simulink library "casper_library_scopes"  (Simulink 8.0)
settings: Solver=ode45  SolverMode=SingleTasking  StartTime=0.0  StopTime=10.0  RelTol=1e-3
libraries: xbsIndex_r4 x476, xps_library x33, casper_library_misc x13, casper_library_scopes x5, casper_library_flow_control x1, simulink x1
(part 1 of 5)
settings Model: Creator=mdexter  LastModifiedBy=paulp

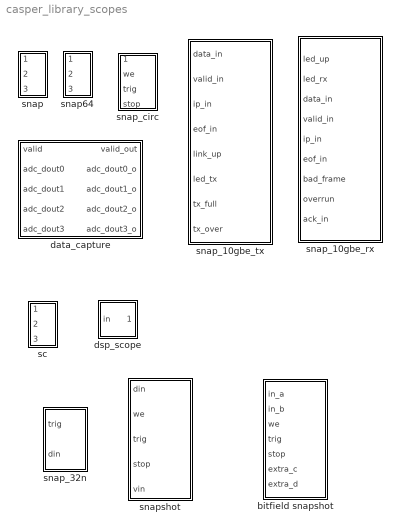
== system casper_library_scopes ==
  bitfield snapshot : Subsystem  Tag=casper:bitsnap  mask(bitsnap){io_names=[a b], io_widths=[16 1], io_bps=[14 0], io_types=[0 2], show_format=on, snap_storage=bram, snap_dram_dimm=2, snap_dram_clock=250, snap_nsamples=10, snap_data_width=32, snap_offset=on, snap_circap=on, snap_value=on, snap_use_dsp48=on, snap_delay=0, extra_names=[c d], extra_widths=[30 2], extra_bps=[0 0], extra_types=[0 0]}
      mask prompts: io_names "Names [msb...lsb]"; io_widths "Bitwidths [msb...lsb]"; io_bps "Binary pts [msb...lsb]"; io_types "Data types [msb...lsb], ufix=0, fix=1, bool=2"; show_format "Print format string?"; snap_storage "Storage medium"; snap_dram_dimm "DRAM dimm"; snap_dram_clock "DRAM clock rate"; snap_nsamples "Number of Samples (2^?)"; snap_data_width "Data width"; snap_offset "Start delay support"; snap_circap "Circular capture support"; snap_value "Extra value capture support"; snap_use_dsp48 "Use DSP48s to implement counters"; snap_delay "Pre-snapshot delay"; extra_names "Names [msb...lsb]"; extra_widths "Widths [msb...lsb]"; extra_bps "Binary pts [msb...lsb]"; extra_types "Data types [msb...lsb], ufix=0, fix=1, bool=2"
      mask help:
      | A wrapped snapshot block. Allows specification of inputs to a snapblock word so the toolflow can automatically set up the scope.
      | See documentation for snapshot for explanation of parameters.
      mask init:
      | bitsnap_init(gcb);
      settings: AttributesFormatString=snap(2):uf16.14,b\nextra(2):uf30.0,uf2.0
      mask TypeOptions snap_storage: bram | dram
      mask Callback snap_storage: bitsnap_callback();
      mask TypeOptions snap_dram_dimm: 1 | 2 | 3 | 4
      mask TypeOptions snap_dram_clock: 200 | 250 | 266 | 300 | 333
      mask TypeOptions snap_data_width: 8 | 16 | 32 | 64 | 128
      mask Callback snap_value: bitsnap_callback();
  data_capture : Subsystem  mask(data_capture){stream_name=adc_dout, nsimult_streams=4}
      mask prompts: stream_name "Stream Name"; nsimult_streams "Number Of Simultaneous Streams"
      mask help:
      | This block is useful for capturing parallel data streams
      | simultaneously and sending the data in structures for analysis
      | using MATLAB.  It is intended as a partial replacement for the
      | Simulink scope block when used with the functions in data_capture_tools.
      |
      | The block does not alter the data at all and costs no hardware
      | because it is purely a simulation block.  The block's Simulink
      | outputs are exactly the same as its inputs with no delay.
      mask init:
      | data_capture_init(gcb, ...
      |     'stream_name', stream_name, ...
      |     'nsimult_streams', nsimult_streams);
  dsp_scope : Subsystem  mask(dsp_scope){n_inputs=4, slice_width=18, bin_pt=17, arith_type=1}
      mask prompts: n_inputs "Number of inputs"; slice_width "Width of each input"; bin_pt "Output Binary Point"; arith_type "Output Arithmetic Type (0=Unsigned, 1 = Signed)"
      mask help:
      | This block provides a convenient interface to plotting waveforms
      | of blocks with serial data output in parallel.  The core example
      | is of the ADC, which outputs 8 samples / clock.  This scope (simulation only)
      | samples sufficently fast (based on the number of parallel inputs)
      | to serialize the output for view in a standard simulink scope.
      |
      | The input must be concatenated parallel data streams, and
      | each data binary point must be 0.  The easiest way to do this is
      | to push  all the inputs through a "cram" block from the
      | GAVRT blockset.
      | easy
      mask init:
      | dsp_scope_init(gcb, ...
      |     'n_inputs', n_inputs, ...
      |     'slice_width', slice_width, ...
      |     'bin_pt', bin_pt, ...
      |     'arith_type', arith_type);
  sc : Subsystem  mask(sc){nsamples=11, offset=0}
      mask prompts: nsamples "No. of samples(2^?)"; offset "Parallel Bus Offset"
      mask help:
      | The 'sc' block is a modified version of the 'snap' block in
      | the same library.  The modification intends to move the software
      | register which has partial control over the 'we' line to the
      | bram as an external port so that multiple brams can use the same
      | gated write enable, i.e. they can share the software register
      | that enables writing to the bram.  This will simplify synchronous writing
      | to multiple brams.
      |
      | The 'sc' core is used in the 'snap_32n' block to mask the
      | 32-bit word limitation of the bram.
      mask init:
      | deprecation_warning('the sc block is to be removed from the casper library, please use the snapshot block instead', 'sc');
      settings: CopyFcn=deprecation_warning('the sc block is to be removed from the casper library, please use the snapshot block instead', 'sc')
      mask Help: eval('xlWeb(''http://casper.berkeley.edu/wiki/Snap'')')
  snap : Subsystem  mask(snap){nsamples=11}
      mask prompts: nsamples "No. of samples(2^?)"
      mask help:
      | The <i>snap</i> block provides a packaged solution to capturing data from
      | the FPGA fabric and making it accessible from the CPU.  The block comes in
      | 2 flavors: <i>snap</i> (which captures to a 32 bit wide Shared BRAM), and
      | <i>snap64</i> (which captures to 2x32 bit wide Shared BRAMs to effect a
      | 64 bit capture).
      mask init:
      | deprecation_warning('the snap block is to be removed from the casper library, please use the snapshot block instead', 'snap');
      settings: CopyFcn=deprecation_warning('the snap block is to be removed from the casper library, please use the snapshot block instead', 'snap')
      mask Help: eval('xlWeb(''http://casper.berkeley.edu/wiki/Snap'')')
  snap64 : Subsystem  mask(snap64){nsamples=11}
      mask prompts: nsamples "No. of samples(2^?)"
      mask help:
      | The <i>snap</i> block provides a packaged solution to capturing data from
      | the FPGA fabric and making it accessible from the CPU.  The block comes in
      | 2 flavors: <i>snap</i> (which captures to a 32 bit wide Shared BRAM), and
      | <i>snap64</i> (which captures to 2x32 bit wide Shared BRAMs to effect a
      | 64 bit capture).
      mask init:
      | deprecation_warning('the snap64 block is to be removed from the casper library, please use the snapshot block instead', 'snap64');
      settings: CopyFcn=deprecation_warning('the snap64 block is to be removed from the casper library, please use the snapshot block instead', 'snap64')
      mask Help: eval('xlWeb(''http://casper.berkeley.edu/wiki/Snap'')')
  snap_10gbe_rx : Subsystem  mask(snap_10gbe_rx){nsamples=11}
      mask prompts: nsamples "No. of samples(2^?)"
      mask help:
      | This snap block provides a packaged solution to capturing a 10GbE datastream from the FPGA fabric and making it accessible from the CPU.  The block captures data in 3 32-bit brams, two for the main data stream and one for out-of-band data (IP addresses, link status, buffer overflow warnings etc).
      |
      | There are two versions, one tailored for RX data streams and one tailored for TX data streams.
      mask init:
      | deprecation_warning('the snap_10gbe_rx block is to be removed from the casper library, please use the snapshot block instead', 'snap_10gbe_rx');
      settings: CopyFcn=deprecation_warning('the snap_10gbe_rx block is to be removed from the casper library, please use the snapshot block instead', 'snap_10gbe_rx')
  snap_10gbe_tx : Subsystem  mask(snap_10gbe_tx){nsamples=11}
      mask prompts: nsamples "No. of samples(2^?)"
      mask help:
      | This snap block provides a packaged solution to capturing a 10GbE datastream from the FPGA fabric and making it accessible from the CPU.  The block captures data in 3 32-bit brams, two for the main data stream and one for out-of-band data (IP addresses, link status, buffer overflow warnings etc).
      |
      | There are two versions, one tailored for RX data streams and one tailored for TX data streams.
      mask init:
      | deprecation_warning('the snap_10gbe_tx block is to be removed from the casper library, please use the snapshot block instead', 'snap_10gbe_tx');
      settings: CopyFcn=deprecation_warning('the snap_10gbe_tx block is to be removed from the casper library, please use the snapshot block instead', 'snap_10gbe_tx')
  snap_32n : Subsystem  mask(snap_32n){nsamples=11, width=4}
      mask prompts: nsamples "Number of Samples (2^"; width "Input Bus Width (32x"
      mask help:
      | Like the snap64 block, this block contains multiple sub-cores
      | that each have a separate bram.  The purpose is to be able to
      | extend the functionality of the 'snap' and 'sc' blocks to beyond
      | the 32-bit word limitation of a single bram by synchronously
      | writing different parts of a larger bus to separate BRAMs.  UNLIKE
      | the snap64 block, the bus width on the 'snap_32n' block is
      | parameterizable to any multiple of 32.
      mask init:
      | deprecation_warning('The snap_32n block is to be removed from the casper library, please use the snapshot block instead', 'snap_32n');
      | snap_32n_init(gcb, ...
      |     'nsamples', nsamples, ...
      |     'width', width);
      settings: CopyFcn=deprecation_warning('the snap_32n block is to be removed from the casper library, please use the snapshot block instead', 'snap_32n')
  snap_circ : Subsystem  mask(snap_circ){nsamples=10}
      mask prompts: nsamples "Number of Samples (2^?)"
      mask help:
      | Backwards compatible with the normal snap block, but with the following upgrades:
      |  1) Ability to offset the trigger. Optionally delay the fabric trigger by a user-specified number of valids.
      |  2) 'Addr' register's MSb now indicates 'busy capturing'.
      |  3) Ability to capture continuously until a stop pulse is received. Data is captured into BRAM continuously, with old data being overwritten until a stop command is received. Then stop capturing when memory is filled. This enables you to get some data before and some data after the stop pulse. Use the 'tr_en_cnt' register to determine where you are in your vector.
      mask init:
      | deprecation_warning('the snap_circ block is to be removed from the casper library, please use the snapshot block instead', 'snap_circ');
      settings: CopyFcn=deprecation_warning('the snap_circ block is to be removed from the casper library, please use the snapshot block instead', 'snap_circ')
  snapshot : Subsystem  Tag=casper:snapshot  mask(snapshot){storage=bram, dram_dimm=1, dram_clock=200, nsamples=10, data_width=32, offset=on, circap=on, value=on, use_dsp48=on}
      mask prompts: storage "Storage medium"; dram_dimm "DRAM dimm"; dram_clock "DRAM clock rate"; nsamples "Number of Samples (2^?)"; data_width "Data width"; offset "Start delay support"; circap "Circular capture support"; value "Extra value capture support"; use_dsp48 "Use DSP48s to implement counters"
      mask help:
      | Standard snap block, but with the following optional extras;
      |  1) Optionally delay the fabric trigger by a user-specified number of valids.
      |  2) Capture continuously after a trigger until a stop pulse is received. Data is captured into BRAM continuously, with old data being overwritten until a stop command is received. Then stop capturing when memory is filled. This enables you to get some data before and some data after the stop pulse. Use the 'tr_en_cnt' register to determine where you are in your vector. 'Addr' register's MSb now indicates 'busy capturing'.
      |  3) Optionally capture a value on an input port to a register at the same time as the first data sample.
      |  4) Implement counters using DSP48Es to save resources.
      mask init:
      | snapshot_init(gcb, ...
      |     'storage', storage, ...
      |     'dram_dimm', dram_dimm, ...
      |     'dram_clock', dram_clock, ...
      |     'nsamples', nsamples, ...
      |     'data_width', data_width, ...
      |     'offset', offset, ...
      |     'circap', circap, ...
      |     'value', value, ...
      |     'use_dsp48', use_dsp48);
      mask TypeOptions storage: bram | dram
      mask Callback storage: snapshot_callback();
      mask TypeOptions dram_dimm: 1 | 2 | 3 | 4
      mask TypeOptions dram_clock: 200 | 250 | 266 | 300 | 333
      mask TypeOptions data_width: 8 | 16 | 32 | 64 | 128

== system casper_library_scopes/bitfield snapshot ==
  in_a : Inport
  in_b : Inport  Port=2
  we : Inport  Port=3
  trig : Inport  Port=4
  stop : Inport  Port=5
  extra_c : Inport  Port=6
  extra_d : Inport  Port=7
  assert_a : xbsIndex_r4/Assert  assert_type=on  type_source=Explicitly  gui_display_data_type=Fixed-point  arith_type=Unsigned  n_bits=16  bin_pt=14  preci_type=Single  exp_width=8  frac_width=24  assert_rate=off  rate_source=Explicitly  period=1  output_port=on  block_type=assert
  assert_b : xbsIndex_r4/Assert  assert_type=on  type_source=Explicitly  gui_display_data_type=Boolean  arith_type=Boolean  n_bits=1  bin_pt=0  preci_type=Single  exp_width=8  frac_width=24  assert_rate=off  rate_source=Explicitly  period=1  output_port=on  block_type=assert
  assextra_c : xbsIndex_r4/Assert  assert_type=on  type_source=Explicitly  gui_display_data_type=Fixed-point  arith_type=Unsigned  n_bits=30  bin_pt=0  preci_type=Single  exp_width=8  frac_width=24  assert_rate=off  rate_source=Explicitly  period=1  output_port=on  block_type=assert
  assextra_d : xbsIndex_r4/Assert  assert_type=on  type_source=Explicitly  gui_display_data_type=Fixed-point  arith_type=Unsigned  n_bits=2  bin_pt=0  preci_type=Single  exp_width=8  frac_width=24  assert_rate=off  rate_source=Explicitly  period=1  output_port=on  block_type=assert
  buscreate : Subsystem  AncestorBlock=casper_library_flow_control/bus_create  mask(bus_create){inputNum=2}
      mask prompts: inputNum "Number of inputs:"
      mask init:
      | bus_create_init(gcb,...
      |     'inputNum', inputNum);
  extracast : xbsIndex_r4/Convert  gui_display_data_type=Fixed-point  arith_type=Unsigned  n_bits=32  bin_pt=0  float_type=Single  exp_bits=8  fraction_bits=24  quantization=Truncate  overflow=Wrap  en=off  latency=0  dbl_ovrd=off  pipeline=off  block_type=convert
  extracreate : Subsystem  AncestorBlock=casper_library_flow_control/bus_create  mask(bus_create){inputNum=2}
      mask prompts: inputNum "Number of inputs:"
      mask init:
      | bus_create_init(gcb,...
      |     'inputNum', inputNum);
  ss : Subsystem  Tag=casper:snapshot  AncestorBlock=casper_library_scopes/snapshot  mask(snapshot){storage=bram, dram_dimm=2, dram_clock=250, nsamples=10, data_width=32, offset=on, circap=on, value=on, use_dsp48=on}
      mask prompts: storage "Storage medium"; dram_dimm "DRAM dimm"; dram_clock "DRAM clock rate"; nsamples "Number of Samples (2^?)"; data_width "Data width"; offset "Start delay support"; circap "Circular capture support"; value "Extra value capture support"; use_dsp48 "Use DSP48s to implement counters"
      mask help:
      | Standard snap block, but with the following optional extras;
      |  1) Optionally delay the fabric trigger by a user-specified number of valids.
      |  2) Capture continuously after a trigger until a stop pulse is received. Data is captured into BRAM continuously, with old data being overwritten until a stop command is received. Then stop capturing when memory is filled. This enables you to get some data before and some data after the stop pulse. Use the 'tr_en_cnt' register to determine where you are in your vector. 'Addr' register's MSb now indicates 'busy capturing'.
      |  3) Optionally capture a value on an input port to a register at the same time as the first data sample.
      |  4) Implement counters using DSP48Es to save resources.
      mask init: same as casper_library_scopes/snapshot
      mask TypeOptions storage: bram | dram
      mask Callback storage: snapshot_callback();
      mask TypeOptions dram_dimm: 1 | 2 | 3 | 4
      mask TypeOptions dram_clock: 200 | 250 | 266 | 300 | 333
      mask TypeOptions data_width: 8 | 16 | 32 | 64 | 128
  wires:
  buscreate/1(bus_out) -> ss/1(din)
  in_a/1 -> assert_a/1
  assert_a/1 -> buscreate/1(in1)
  in_b/1 -> assert_b/1
  assert_b/1 -> buscreate/2(in2)
  we/1 -> ss/2(we)
  trig/1 -> ss/3(trig)
  stop/1 -> ss/4(stop)
  extracreate/1(bus_out) -> extracast/1
  extracast/1 -> ss/5(vin)
  extra_c/1 -> assextra_c/1
  assextra_c/1 -> extracreate/1(in1)
  extra_d/1 -> assextra_d/1
  assextra_d/1 -> extracreate/2(in2)

== system casper_library_scopes/data_capture ==
  valid : Inport
  adc_dout0 : Inport  Port=2
  adc_dout1 : Inport  Port=3
  adc_dout2 : Inport  Port=4
  adc_dout3 : Inport  Port=5
  ToWorkspace_adc_dout0 : ToWorkspace  VariableName=adc_dout0  SampleTime=-1  SaveFormat=Structure
  ToWorkspace_adc_dout1 : ToWorkspace  VariableName=adc_dout1  SampleTime=-1  SaveFormat=Structure
  ToWorkspace_adc_dout2 : ToWorkspace  VariableName=adc_dout2  SampleTime=-1  SaveFormat=Structure
  ToWorkspace_adc_dout3 : ToWorkspace  VariableName=adc_dout3  SampleTime=-1  SaveFormat=Structure
  ToWorkspace_valid : ToWorkspace  VariableName=adc_dout_valid  SampleTime=-1  SaveFormat=Structure
  valid_out : Outport
  adc_dout0_o : Outport  Port=2
  adc_dout1_o : Outport  Port=3
  adc_dout2_o : Outport  Port=4
  adc_dout3_o : Outport  Port=5
  wires:
  adc_dout3/1 -> adc_dout3_o/1, ToWorkspace_adc_dout3/1
  adc_dout2/1 -> adc_dout2_o/1, ToWorkspace_adc_dout2/1
  adc_dout1/1 -> adc_dout1_o/1, ToWorkspace_adc_dout1/1
  adc_dout0/1 -> adc_dout0_o/1, ToWorkspace_adc_dout0/1
  valid/1 -> valid_out/1, ToWorkspace_valid/1

== system casper_library_scopes/dsp_scope ==
  in : Inport
  bus_expand : casper_library_flow_control/bus_expand  mode=divisions of equal size  outputNum=4  outputWidth=18  outputBinaryPt=17  outputArithmeticType=1  show_format=off  outputToWorkspace=off  variablePrefix=out  outputToModelAsWell=on
      settings: AttributesFormatString=4 outputs
  sel : simulink/Sources/Counter Free-Running  NumBits=2  tsamp=0.25
  switch : MultiPortSwitch  DataPortOrder=Zero-based contiguous  Inputs=4  zeroidx=on
  out : Outport
  wires:
  in/1 -> bus_expand/1
  switch/1 -> out/1
  sel/1 -> switch/1
  bus_expand/1 -> switch/2
  bus_expand/2 -> switch/3
  ? -> switch/4
  ? -> switch/5

== system casper_library_scopes/sc ==
  din : Inport
  trig : Inport  Port=2
  read_freeze : Inport  Port=3
  Constant : xbsIndex_r4/Constant  const=2^nsamples  gui_display_data_type=Fixed-point  arith_type=Unsigned  n_bits=32  bin_pt=0  preci_type=Single  exp_width=8  frac_width=24  explicit_period=on  period=1  equ=P=C  opselect=C  inp2=PCIN>>17  opr=+  inp1=P  carry=CIN  dbl_ovrd=off  block_type=constant
  Counter : xbsIndex_r4/Counter  cnt_type=Count Limited  cnt_to=Inf  operation=Up  start_count=0  cnt_by_val=1  arith_type=Unsigned  n_bits=nsamples+1  bin_pt=0  load_pin=off  rst=on  en=off  explicit_period=on  period=1  dbl_ovrd=off  use_behavioral_HDL=off  implementation=Fabric  use_rpm=off  block_type=counter
  Inverter : xbsIndex_r4/Inverter  en=off  latency=0  dbl_ovrd=off  block_type=inv
  Logical : xbsIndex_r4/Logical  logical_function=AND  inputs=2  en=off  latency=0  precision=Full  arith_type=Unsigned  n_bits=16  bin_pt=0  align_bp=on  dbl_ovrd=off  block_type=logical
  Reinterpret : xbsIndex_r4/Reinterpret  force_arith_type=on  arith_type=Unsigned  force_bin_pt=on  bin_pt=0  block_type=reinterpret
      settings: infoedit="Changes signal type without altering the binary representation.   You can changed the signal between signed and unsigned, and relocate the binary point.<P><P>Hardware notes: In hardware this block costs nothing.<P><P>Example:  Suppose the input is 6 bits wide, signed, with 2 fractional bits, and the output is forced to unsigned with 0 fractional bits.  Then an input of -2.0 (1110.00 in binary 2's complement) becomes an output of 56 (111000 in binary)."  block_version=10.1.1
  Relational : xbsIndex_r4/Relational  mode=a<b  en=off  latency=1  dbl_ovrd=off  block_type=relational
      settings: block_version=10.1.3
  Slice : xbsIndex_r4/Slice  nbits=1  boolean_output=on  mode=Lower Bit Location + Width  bit1=0  base1=MSB of Input  bit0=0  base0=LSB of Input  dbl_ovrd=off  block_type=slice
      settings: infoedit="Extracts a given range of bits from each input sample and presents it at the output.  The output type is ordinarily unsigned with binary point at zero, but can be Boolean when the slice is one bit wide.<P><P>Hardware notes: In hardware this block costs nothing."  block_version=10.1.3
  bram : xps_library/Shared BRAM  Tag=xps:bram  arith_type=Unsigned  addr_width=nsamples  data_width=32  reg_prim_output=on  reg_core_output=on  optimization=Minimum_Area  data_bin_pt=0  init_vals=0  sample_rate=1
  data_sl : xbsIndex_r4/Slice  nbits=32  boolean_output=off  mode=Lower Bit Location + Width  bit1=0  base1=MSB of Input  bit0=offset  base0=LSB of Input  dbl_ovrd=off  block_type=slice
      settings: infoedit="Extracts a given range of bits from each input sample and presents it at the output.  The output type is ordinarily unsigned with binary point at zero, but can be Boolean when the slice is one bit wide.<P><P>Hardware notes: In hardware this block costs nothing."  block_version=10.1.3
  wires:
  data_sl/1 -> Reinterpret/1
  Constant/1 -> Relational/2
  Relational/1 -> bram/3
  read_freeze/1 -> Slice/1
  Slice/1 -> Inverter/1
  Logical/1 -> Counter/1
  Inverter/1 -> Logical/2
  trig/1 -> Logical/1
  Counter/1 -> Relational/1, bram/1
  Reinterpret/1 -> bram/2
  din/1 -> data_sl/1

== system casper_library_scopes/snap ==
  din : Inport
  trig : Inport  Port=2
  we : Inport  Port=3
  Constant : xbsIndex_r4/Constant  const=1  gui_display_data_type=Fixed-point  arith_type=Boolean  n_bits=1  bin_pt=0  preci_type=Single  exp_width=8  frac_width=24  explicit_period=on  period=1  equ=P=C  opselect=C  inp2=PCIN>>17  opr=+  inp1=P  carry=CIN  dbl_ovrd=off  block_type=constant
      settings: block_version=10.1.1
  Constant1 : xbsIndex_r4/Constant  const=1  gui_display_data_type=Fixed-point  arith_type=Boolean  n_bits=1  bin_pt=0  preci_type=Single  exp_width=8  frac_width=24  explicit_period=on  period=1  equ=P=C  opselect=C  inp2=PCIN>>17  opr=+  inp1=P  carry=CIN  dbl_ovrd=off  block_type=constant
      settings: block_version=10.1.1
  Constant13 : Constant
  Constant2 : xbsIndex_r4/Constant  const=1  gui_display_data_type=Fixed-point  arith_type=Boolean  n_bits=1  bin_pt=0  preci_type=Single  exp_width=8  frac_width=24  explicit_period=on  period=1  equ=P=C  opselect=C  inp2=PCIN>>17  opr=+  inp1=P  carry=CIN  dbl_ovrd=off  block_type=constant
      settings: block_version=10.1.1
  Inverter : xbsIndex_r4/Inverter  en=off  latency=0  dbl_ovrd=off  block_type=inv
      settings: xl_area=[0, 0, 0, 0, 0, 0, 0]  block_version=10.1.1
  Logical1 : xbsIndex_r4/Logical  logical_function=AND  inputs=2  en=off  latency=0  precision=Full  arith_type=Unsigned  n_bits=8  bin_pt=2  align_bp=on  dbl_ovrd=off  block_type=logical
      settings: xl_area=[0, 0, 0, 0, 0, 0, 0]  block_version=10.1.1
  Mux1 : xbsIndex_r4/Mux  inputs=2  en=off  latency=0  precision=Full  arith_type="Signed  (2's comp)"  n_bits=8  bin_pt=2  quantization=Truncate  overflow=Wrap  dbl_ovrd=off  block_type=mux
      settings: xl_area=[0, 0, 0, 0, 0, 0, 0]  block_version=10.1.1
  Mux2 : xbsIndex_r4/Mux  inputs=2  en=off  latency=0  precision=Full  arith_type="Signed  (2's comp)"  n_bits=8  bin_pt=2  quantization=Truncate  overflow=Wrap  dbl_ovrd=off  block_type=mux
      settings: xl_area=[0, 0, 0, 0, 0, 0, 0]  block_version=10.1.1
  Register : xbsIndex_r4/Register  init=0  rst=on  en=on  dbl_ovrd=off  block_type=register
      settings: xl_area=[0, 0, 0, 0, 0, 0, 0]  block_version=10.1.1
  Register1 : xbsIndex_r4/Register  init=0  rst=on  en=on  dbl_ovrd=off  block_type=register
      settings: xl_area=[0, 0, 0, 0, 0, 0, 0]  block_version=10.1.1
  Reinterpret : xbsIndex_r4/Reinterpret  force_arith_type=on  arith_type=Unsigned  force_bin_pt=on  bin_pt=0  block_type=reinterpret
      settings: infoedit="Changes signal type without altering the binary representation.   You can changed the signal between signed and unsigned, and relocate the binary point.<P><P>Hardware notes: In hardware this block costs nothing.<P><P>Example:  Suppose the input is 6 bits wide, signed, with 2 fractional bits, and the output is forced to unsigned with 0 fractional bits.  Then an input of -2.0 (1110.00 in binary 2's complement) becomes an output of 56 (111000 in binary)."  block_version=10.1.1
  addr : xps_library/software register  Tag=xps:sw_reg  numios=1  io_dir=To Processor  io_delay=0  sample_period=1  name1=reg  bitwidth1=32  arith_type1=Unsigned  bin_pt1=0
  bram : xps_library/Shared BRAM  Tag=xps:bram  arith_type=Unsigned  addr_width=nsamples  data_width=32  reg_prim_output=on  reg_core_output=on  optimization=Minimum_Area  data_bin_pt=0  init_vals=0  sample_rate=1
  ctrl : xps_library/software register  Tag=xps:sw_reg  numios=1  io_dir=From Processor  io_delay=0  sample_period=1  name1=reg  bitwidth1=32  arith_type1=Unsigned  bin_pt1=0
  enable : xbsIndex_r4/Slice  nbits=1  boolean_output=on  mode=Lower Bit Location + Width  bit1=0  base1=LSB of Input  bit0=0  base0=LSB of Input  dbl_ovrd=off  block_type=slice
      settings: infoedit="Extracts a given range of bits from each input sample and presents it at the output.  The output type is ordinarily unsigned with binary point at zero, but can be Boolean when the slice is one bit wide.<P><P>Hardware notes: In hardware this block costs nothing."  block_version=10.1.1
  freeze_cntr : casper_library_misc/freeze_cntr  CounterBits=nsamples
  posedge : casper_library_misc/edge_detect  edge=Rising  polarity=Active High  x_in=[0 0.08 0.08 0.16 0.16 0.24 0.24 0.32 0.32 0.4]  y_in="[-1 -1  1  1  1  1  1  1  1  1]"  x_out=[0.6 0.68 0.68 0.76 0.76 0.84 0.84 0.92 0.92 1]  y_out="[-1 -1  1  1 -1 -1 -1 -1 -1 -1]"
  trig1 : xbsIndex_r4/Slice  nbits=1  boolean_output=on  mode=Lower Bit Location + Width  bit1=0  base1=LSB of Input  bit0=1  base0=LSB of Input  dbl_ovrd=off  block_type=slice
      settings: infoedit="Extracts a given range of bits from each input sample and presents it at the output.  The output type is ordinarily unsigned with binary point at zero, but can be Boolean when the slice is one bit wide.<P><P>Hardware notes: In hardware this block costs nothing."  block_version=10.1.1
  valid : xbsIndex_r4/Slice  nbits=1  boolean_output=on  mode=Lower Bit Location + Width  bit1=0  base1=LSB of Input  bit0=2  base0=LSB of Input  dbl_ovrd=off  block_type=slice
      settings: infoedit="Extracts a given range of bits from each input sample and presents it at the output.  The output type is ordinarily unsigned with binary point at zero, but can be Boolean when the slice is one bit wide.<P><P>Hardware notes: In hardware this block costs nothing."  block_version=10.1.1
  wires:
  Mux2/1 -> Logical1/1
  Inverter/1 -> Logical1/2
  Logical1/1 -> Register/2
  valid/1 -> Mux1/1
  trig1/1 -> Mux2/1
  Register1/1 -> addr/1
  Constant2/1 -> Mux1/3
  we/1 -> Mux1/2
  Mux1/1 -> freeze_cntr/1
  Constant1/1 -> Mux2/3
  Constant/1 -> Register/1
  posedge/1 -> Inverter/1, Register1/2, Register/3
  ctrl/1 -> trig1/1, valid/1, enable/1
  din/1 -> Reinterpret/1
  Reinterpret/1 -> bram/2
  Constant13/1 -> ctrl/1
  freeze_cntr/2 -> Register1/3, bram/3
  Register/1 -> freeze_cntr/2
  enable/1 -> posedge/1
  freeze_cntr/1 -> bram/1, Register1/1
  trig/1 -> Mux2/2

== system casper_library_scopes/snap64 ==
  din : Inport
  trig : Inport  Port=2
  we : Inport  Port=3
  Constant : xbsIndex_r4/Constant  const=1  gui_display_data_type=Fixed-point  arith_type=Boolean  n_bits=1  bin_pt=0  preci_type=Single  exp_width=8  frac_width=24  explicit_period=on  period=1  equ=P=C  opselect=C  inp2=PCIN>>17  opr=+  inp1=P  carry=CIN  dbl_ovrd=off  block_type=constant
      settings: block_version=10.1.1
  Constant1 : xbsIndex_r4/Constant  const=1  gui_display_data_type=Fixed-point  arith_type=Boolean  n_bits=1  bin_pt=0  preci_type=Single  exp_width=8  frac_width=24  explicit_period=on  period=1  equ=P=C  opselect=C  inp2=PCIN>>17  opr=+  inp1=P  carry=CIN  dbl_ovrd=off  block_type=constant
      settings: block_version=10.1.1
  Constant13 : Constant
  Constant2 : xbsIndex_r4/Constant  const=1  gui_display_data_type=Fixed-point  arith_type=Boolean  n_bits=1  bin_pt=0  preci_type=Single  exp_width=8  frac_width=24  explicit_period=on  period=1  equ=P=C  opselect=C  inp2=PCIN>>17  opr=+  inp1=P  carry=CIN  dbl_ovrd=off  block_type=constant
      settings: block_version=10.1.1
  Inverter : xbsIndex_r4/Inverter  en=off  latency=0  dbl_ovrd=off  block_type=inv
      settings: xl_area=[0, 0, 0, 0, 0, 0, 0]  block_version=10.1.1
  Logical1 : xbsIndex_r4/Logical  logical_function=AND  inputs=2  en=off  latency=0  precision=Full  arith_type=Unsigned  n_bits=8  bin_pt=2  align_bp=on  dbl_ovrd=off  block_type=logical
      settings: xl_area=[0, 0, 0, 0, 0, 0, 0]  block_version=10.1.1
  Mux1 : xbsIndex_r4/Mux  inputs=2  en=off  latency=0  precision=Full  arith_type="Signed  (2's comp)"  n_bits=8  bin_pt=2  quantization=Truncate  overflow=Wrap  dbl_ovrd=off  block_type=mux
      settings: xl_area=[0, 0, 0, 0, 0, 0, 0]  block_version=10.1.1
  Mux2 : xbsIndex_r4/Mux  inputs=2  en=off  latency=0  precision=Full  arith_type="Signed  (2's comp)"  n_bits=8  bin_pt=2  quantization=Truncate  overflow=Wrap  dbl_ovrd=off  block_type=mux
      settings: xl_area=[0, 0, 0, 0, 0, 0, 0]  block_version=10.1.1
  Register : xbsIndex_r4/Register  init=0  rst=on  en=on  dbl_ovrd=off  block_type=register
      settings: xl_area=[0, 0, 0, 0, 0, 0, 0]  block_version=10.1.1
  Register1 : xbsIndex_r4/Register  init=0  rst=on  en=on  dbl_ovrd=off  block_type=register
      settings: xl_area=[0, 0, 0, 0, 0, 0, 0]  block_version=10.1.1
  Reinterpret3 : xbsIndex_r4/Reinterpret  force_arith_type=on  arith_type=Unsigned  force_bin_pt=on  bin_pt=0  block_type=reinterpret
      settings: infoedit="Changes signal type without altering the binary representation.   You can changed the signal between signed and unsigned, and relocate the binary point.<P><P>Hardware notes: In hardware this block costs nothing.<P><P>Example:  Suppose the input is 6 bits wide, signed, with 2 fractional bits, and the output is forced to unsigned with 0 fractional bits.  Then an input of -2.0 (1110.00 in binary 2's complement) becomes an output of 56 (111000 in binary)."  block_version=10.1.1
  addr : xps_library/software register  Tag=xps:sw_reg  numios=1  io_dir=To Processor  io_delay=0  sample_period=1  name1=reg  bitwidth1=32  arith_type1=Unsigned  bin_pt1=0
  bram_lsb : xps_library/Shared BRAM  Tag=xps:bram  arith_type=Unsigned  addr_width=nsamples  data_width=32  reg_prim_output=on  reg_core_output=on  optimization=Minimum_Area  data_bin_pt=0  init_vals=0  sample_rate=1
  bram_msb : xps_library/Shared BRAM  Tag=xps:bram  arith_type=Unsigned  addr_width=nsamples  data_width=32  reg_prim_output=on  reg_core_output=on  optimization=Minimum_Area  data_bin_pt=0  init_vals=0  sample_rate=1
  ctrl : xps_library/software register  Tag=xps:sw_reg  numios=1  io_dir=From Processor  io_delay=0  sample_period=1  name1=reg  bitwidth1=32  arith_type1=Unsigned  bin_pt1=0
  en1 : xbsIndex_r4/Slice  nbits=32  boolean_output=off  mode=Lower Bit Location + Width  bit1=0  base1=LSB of Input  bit0=32  base0=LSB of Input  dbl_ovrd=off  block_type=slice
      settings: infoedit="Extracts a given range of bits from each input sample and presents it at the output.  The output type is ordinarily unsigned with binary point at zero, but can be Boolean when the slice is one bit wide.<P><P>Hardware notes: In hardware this block costs nothing."  block_version=10.1.1
  en2 : xbsIndex_r4/Slice  nbits=32  boolean_output=off  mode=Lower Bit Location + Width  bit1=0  base1=LSB of Input  bit0=0  base0=LSB of Input  dbl_ovrd=off  block_type=slice
      settings: infoedit="Extracts a given range of bits from each input sample and presents it at the output.  The output type is ordinarily unsigned with binary point at zero, but can be Boolean when the slice is one bit wide.<P><P>Hardware notes: In hardware this block costs nothing."  block_version=10.1.1
  enable : xbsIndex_r4/Slice  nbits=1  boolean_output=on  mode=Lower Bit Location + Width  bit1=0  base1=LSB of Input  bit0=0  base0=LSB of Input  dbl_ovrd=off  block_type=slice
      settings: infoedit="Extracts a given range of bits from each input sample and presents it at the output.  The output type is ordinarily unsigned with binary point at zero, but can be Boolean when the slice is one bit wide.<P><P>Hardware notes: In hardware this block costs nothing."  block_version=10.1.1
  freeze_cntr : casper_library_misc/freeze_cntr  CounterBits=nsamples
  posedge : casper_library_misc/edge_detect  edge=Rising  polarity=Active High  x_in=[0 0.08 0.08 0.16 0.16 0.24 0.24 0.32 0.32 0.4]  y_in="[-1 -1  1  1  1  1  1  1  1  1]"  x_out=[0.6 0.68 0.68 0.76 0.76 0.84 0.84 0.92 0.92 1]  y_out="[-1 -1  1  1 -1 -1 -1 -1 -1 -1]"
  trig1 : xbsIndex_r4/Slice  nbits=1  boolean_output=on  mode=Lower Bit Location + Width  bit1=0  base1=LSB of Input  bit0=1  base0=LSB of Input  dbl_ovrd=off  block_type=slice
      settings: infoedit="Extracts a given range of bits from each input sample and presents it at the output.  The output type is ordinarily unsigned with binary point at zero, but can be Boolean when the slice is one bit wide.<P><P>Hardware notes: In hardware this block costs nothing."  block_version=10.1.1
  valid : xbsIndex_r4/Slice  nbits=1  boolean_output=on  mode=Lower Bit Location + Width  bit1=0  base1=LSB of Input  bit0=2  base0=LSB of Input  dbl_ovrd=off  block_type=slice
      settings: infoedit="Extracts a given range of bits from each input sample and presents it at the output.  The output type is ordinarily unsigned with binary point at zero, but can be Boolean when the slice is one bit wide.<P><P>Hardware notes: In hardware this block costs nothing."  block_version=10.1.1
  wires:
  freeze_cntr/1 -> bram_lsb/1, bram_msb/1, Register1/1
  Register/1 -> freeze_cntr/2
  Mux2/1 -> Logical1/1
  Inverter/1 -> Logical1/2
  Logical1/1 -> Register/2
  valid/1 -> Mux1/1
  trig1/1 -> Mux2/1
  Register1/1 -> addr/1
  Constant2/1 -> Mux1/3
  we/1 -> Mux1/2
  Mux1/1 -> freeze_cntr/1
  Constant1/1 -> Mux2/3
  Constant/1 -> Register/1
  posedge/1 -> Inverter/1, Register1/2, Register/3
  ctrl/1 -> trig1/1, valid/1, enable/1
  Constant13/1 -> ctrl/1
  freeze_cntr/2 -> bram_lsb/3, bram_msb/3, Register1/3
  enable/1 -> posedge/1
  trig/1 -> Mux2/2
  Reinterpret3/1 -> en1/1, en2/1
  din/1 -> Reinterpret3/1
  en1/1 -> bram_msb/2
  en2/1 -> bram_lsb/2

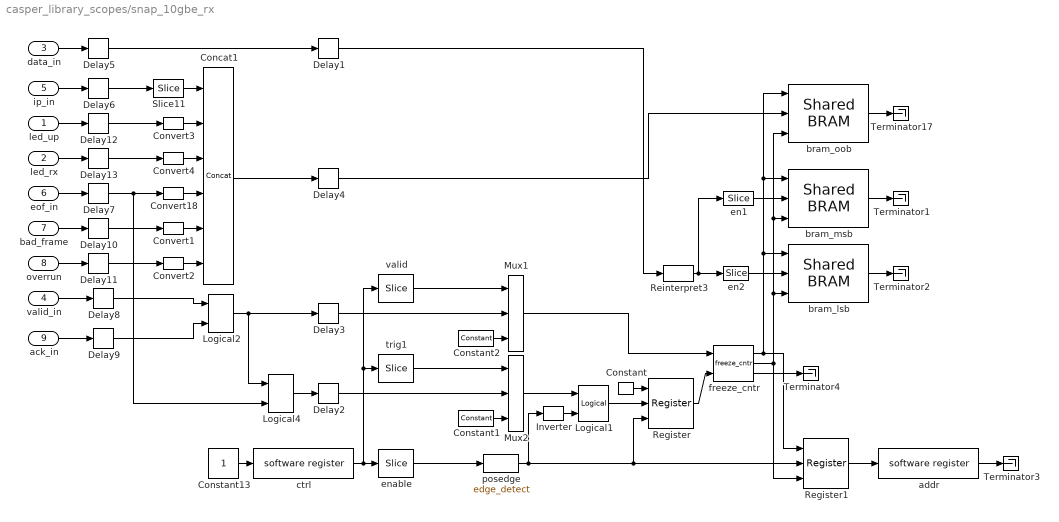
== system casper_library_scopes/snap_10gbe_rx ==
  led_up : Inport
  led_rx : Inport  Port=2
  data_in : Inport  Port=3
  valid_in : Inport  Port=4
  ip_in : Inport  Port=5
  eof_in : Inport  Port=6
  bad_frame : Inport  Port=7
  overrun : Inport  Port=8
  ack_in : Inport  Port=9
  Concat1 : xbsIndex_r4/Concat  num_inputs=6  dbl_ovrd=off  block_type=concat
      settings: block_version=10.1.3
  Constant : xbsIndex_r4/Constant  const=1  gui_display_data_type=Fixed-point  arith_type=Boolean  n_bits=1  bin_pt=0  preci_type=Single  exp_width=8  frac_width=24  explicit_period=on  period=1  equ=P=C  opselect=C  inp2=PCIN>>17  opr=+  inp1=P  carry=CIN  dbl_ovrd=off  block_type=constant
  Constant1 : xbsIndex_r4/Constant  const=1  gui_display_data_type=Fixed-point  arith_type=Boolean  n_bits=1  bin_pt=0  preci_type=Single  exp_width=8  frac_width=24  explicit_period=on  period=1  equ=P=C  opselect=C  inp2=PCIN>>17  opr=+  inp1=P  carry=CIN  dbl_ovrd=off  block_type=constant
  Constant13 : Constant
  Constant2 : xbsIndex_r4/Constant  const=1  gui_display_data_type=Fixed-point  arith_type=Boolean  n_bits=1  bin_pt=0  preci_type=Single  exp_width=8  frac_width=24  explicit_period=on  period=1  equ=P=C  opselect=C  inp2=PCIN>>17  opr=+  inp1=P  carry=CIN  dbl_ovrd=off  block_type=constant
  Convert{1..4,18} (5 alike) : xbsIndex_r4/Convert  gui_display_data_type=Fixed-point  arith_type=Unsigned  n_bits=1  bin_pt=0  float_type=Single  exp_bits=8  fraction_bits=24  quantization=Truncate  overflow=Wrap  en=off  latency=0  dbl_ovrd=off  pipeline=off  block_type=convert
      settings: xl_area=[0, 0, 0, 0, 0, 0, 0]  block_version=10.1.3
  Delay{1..13} (13 alike) : xbsIndex_r4/Delay  rst=off  infoeditControl=Selection of Reset will increase slice count due to use of real FFs and instead of SRLs  en=off  latency=2  dbl_ovrd=off  reg_retiming=on  block_type=delay
      settings: xl_area=[0, 0, 0, 0, 0, 0, 0]
  Inverter : xbsIndex_r4/Inverter  en=off  latency=0  dbl_ovrd=off  block_type=inv
      settings: xl_area=[0, 0, 0, 0, 0, 0, 0]
  Logical1 : xbsIndex_r4/Logical  logical_function=AND  inputs=2  en=off  latency=0  precision=Full  arith_type=Unsigned  n_bits=8  bin_pt=2  align_bp=on  dbl_ovrd=off  block_type=logical
      settings: xl_area=[0, 0, 0, 0, 0, 0, 0]
  Logical2 : xbsIndex_r4/Logical  logical_function=AND  inputs=2  en=off  latency=0  precision=Full  arith_type=Unsigned  n_bits=8  bin_pt=2  align_bp=on  dbl_ovrd=off  block_type=logical
      settings: xl_area=[0, 0, 0, 0, 0, 0, 0]
  Logical4 : xbsIndex_r4/Logical  logical_function=AND  inputs=2  en=off  latency=0  precision=Full  arith_type=Unsigned  n_bits=8  bin_pt=2  align_bp=on  dbl_ovrd=off  block_type=logical
      settings: xl_area=[0, 0, 0, 0, 0, 0, 0]
  Mux1 : xbsIndex_r4/Mux  inputs=2  en=off  latency=0  precision=Full  arith_type="Signed  (2's comp)"  n_bits=8  bin_pt=2  quantization=Truncate  overflow=Wrap  dbl_ovrd=off  block_type=mux
      settings: xl_area=[0, 0, 0, 0, 0, 0, 0]
  Mux2 : xbsIndex_r4/Mux  inputs=2  en=off  latency=0  precision=Full  arith_type="Signed  (2's comp)"  n_bits=8  bin_pt=2  quantization=Truncate  overflow=Wrap  dbl_ovrd=off  block_type=mux
      settings: xl_area=[0, 0, 0, 0, 0, 0, 0]
  Register : xbsIndex_r4/Register  init=0  rst=on  en=on  dbl_ovrd=off  block_type=register
      settings: xl_area=[0, 0, 0, 0, 0, 0, 0]
  Register1 : xbsIndex_r4/Register  init=0  rst=on  en=on  dbl_ovrd=off  block_type=register
      settings: xl_area=[0, 0, 0, 0, 0, 0, 0]
  Reinterpret3 : xbsIndex_r4/Reinterpret  force_arith_type=on  arith_type=Unsigned  force_bin_pt=on  bin_pt=0  block_type=reinterpret
      settings: infoedit="Changes signal type without altering the binary representation.   You can changed the signal between signed and unsigned, and relocate the binary point.<P><P>Hardware notes: In hardware this block costs nothing.<P><P>Example:  Suppose the input is 6 bits wide, signed, with 2 fractional bits, and the output is forced to unsigned with 0 fractional bits.  Then an input of -2.0 (1110.00 in binary 2's complement) becomes an output of 56 (111000 in binary)."  block_version=10.1.3
  Slice11 : xbsIndex_r4/Slice  nbits=32-5  boolean_output=off  mode=Lower Bit Location + Width  bit1=0  base1=MSB of Input  bit0=0  base0=LSB of Input  dbl_ovrd=off  block_type=slice
      settings: infoedit="Extracts a given range of bits from each input sample and presents it at the output.  The output type is ordinarily unsigned with binary point at zero, but can be Boolean when the slice is one bit wide.<P><P>Hardware notes: In hardware this block costs nothing."  block_version=10.1.3
  Terminator{1..4,17} (5 alike) : Terminator
  addr : xps_library/software register  Tag=xps:sw_reg  numios=1  io_dir=To Processor  io_delay=0  sample_period=1  name1=reg  bitwidth1=32  arith_type1=Unsigned  bin_pt1=0
  bram_lsb : xps_library/Shared BRAM  Tag=xps:bram  arith_type=Unsigned  addr_width=nsamples  data_width=32  reg_prim_output=on  reg_core_output=on  optimization=Minimum_Area  data_bin_pt=0  init_vals=0  sample_rate=1
  bram_msb : xps_library/Shared BRAM  Tag=xps:bram  arith_type=Unsigned  addr_width=nsamples  data_width=32  reg_prim_output=on  reg_core_output=on  optimization=Minimum_Area  data_bin_pt=0  init_vals=0  sample_rate=1
  bram_oob : xps_library/Shared BRAM  Tag=xps:bram  arith_type=Unsigned  addr_width=nsamples  data_width=32  reg_prim_output=on  reg_core_output=on  optimization=Minimum_Area  data_bin_pt=0  init_vals=0  sample_rate=1
  ctrl : xps_library/software register  Tag=xps:sw_reg  numios=1  io_dir=From Processor  io_delay=0  sample_period=1  name1=reg  bitwidth1=32  arith_type1=Unsigned  bin_pt1=0
  en1 : xbsIndex_r4/Slice  nbits=32  boolean_output=off  mode=Lower Bit Location + Width  bit1=0  base1=LSB of Input  bit0=32  base0=LSB of Input  dbl_ovrd=off  block_type=slice
      settings: infoedit="Extracts a given range of bits from each input sample and presents it at the output.  The output type is ordinarily unsigned with binary point at zero, but can be Boolean when the slice is one bit wide.<P><P>Hardware notes: In hardware this block costs nothing."  block_version=10.1.3
  en2 : xbsIndex_r4/Slice  nbits=32  boolean_output=off  mode=Lower Bit Location + Width  bit1=0  base1=LSB of Input  bit0=0  base0=LSB of Input  dbl_ovrd=off  block_type=slice
      settings: infoedit="Extracts a given range of bits from each input sample and presents it at the output.  The output type is ordinarily unsigned with binary point at zero, but can be Boolean when the slice is one bit wide.<P><P>Hardware notes: In hardware this block costs nothing."  block_version=10.1.3
  enable : xbsIndex_r4/Slice  nbits=1  boolean_output=on  mode=Lower Bit Location + Width  bit1=0  base1=LSB of Input  bit0=0  base0=LSB of Input  dbl_ovrd=off  block_type=slice
      settings: infoedit="Extracts a given range of bits from each input sample and presents it at the output.  The output type is ordinarily unsigned with binary point at zero, but can be Boolean when the slice is one bit wide.<P><P>Hardware notes: In hardware this block costs nothing."  block_version=10.1.3
  freeze_cntr : casper_library_misc/freeze_cntr  CounterBits=nsamples
  posedge : casper_library_misc/edge_detect  edge=Rising  polarity=Active High  x_in=[0 0.08 0.08 0.16 0.16 0.24 0.24 0.32 0.32 0.4]  y_in="[-1 -1  1  1  1  1  1  1  1  1]"  x_out=[0.6 0.68 0.68 0.76 0.76 0.84 0.84 0.92 0.92 1]  y_out="[-1 -1  1  1 -1 -1 -1 -1 -1 -1]"
  trig1 : xbsIndex_r4/Slice  nbits=1  boolean_output=on  mode=Lower Bit Location + Width  bit1=0  base1=LSB of Input  bit0=1  base0=LSB of Input  dbl_ovrd=off  block_type=slice
      settings: infoedit="Extracts a given range of bits from each input sample and presents it at the output.  The output type is ordinarily unsigned with binary point at zero, but can be Boolean when the slice is one bit wide.<P><P>Hardware notes: In hardware this block costs nothing."  block_version=10.1.3
  valid : xbsIndex_r4/Slice  nbits=1  boolean_output=on  mode=Lower Bit Location + Width  bit1=0  base1=LSB of Input  bit0=2  base0=LSB of Input  dbl_ovrd=off  block_type=slice
      settings: infoedit="Extracts a given range of bits from each input sample and presents it at the output.  The output type is ordinarily unsigned with binary point at zero, but can be Boolean when the slice is one bit wide.<P><P>Hardware notes: In hardware this block costs nothing."  block_version=10.1.3
  wires:
  addr/1 -> Terminator3/1
  freeze_cntr/3 -> Terminator4/1
  bram_lsb/1 -> Terminator2/1
  bram_msb/1 -> Terminator1/1
  bram_oob/1 -> Terminator17/1
  Convert2/1 -> Concat1/6
  Convert1/1 -> Concat1/5
  Convert18/1 -> Concat1/4
  Convert4/1 -> Concat1/3
  Convert3/1 -> Concat1/2
  Slice11/1 -> Concat1/1
  Delay13/1 -> Convert4/1
  led_rx/1 -> Delay13/1
  Delay12/1 -> Convert3/1
  led_up/1 -> Delay12/1
  Delay11/1 -> Convert2/1
  overrun/1 -> Delay11/1
  Delay10/1 -> Convert1/1
  bad_frame/1 -> Delay10/1
  Delay9/1 -> Logical2/2
  Delay8/1 -> Logical2/1
  Delay7/1 -> Logical4/2, Convert18/1
  Delay6/1 -> Slice11/1
  Delay5/1 -> Delay1/1
  Delay3/1 -> Mux1/2
  Delay2/1 -> Mux2/2
  Logical2/1 -> Logical4/1, Delay3/1
  ack_in/1 -> Delay9/1
  eof_in/1 -> Delay7/1
  valid_in/1 -> Delay8/1
  Logical4/1 -> Delay2/1
  Delay4/1 -> bram_oob/2
  Delay1/1 -> Reinterpret3/1
  ip_in/1 -> Delay6/1
  data_in/1 -> Delay5/1
  Concat1/1 -> Delay4/1
  en2/1 -> bram_lsb/2
  en1/1 -> bram_msb/2
  Reinterpret3/1 -> en2/1, en1/1
  enable/1 -> posedge/1
  freeze_cntr/2 -> Register1/3, bram_oob/3, bram_msb/3, bram_lsb/3
  Constant13/1 -> ctrl/1
  ctrl/1 -> enable/1, valid/1, trig1/1
  posedge/1 -> Register/3, Register1/2, Inverter/1
  Constant/1 -> Register/1
  Constant1/1 -> Mux2/3
  Mux1/1 -> freeze_cntr/1
  Constant2/1 -> Mux1/3
  Register1/1 -> addr/1
  trig1/1 -> Mux2/1
  valid/1 -> Mux1/1
  Logical1/1 -> Register/2
  Inverter/1 -> Logical1/2
  Mux2/1 -> Logical1/1
  Register/1 -> freeze_cntr/2
  freeze_cntr/1 -> Register1/1, bram_oob/1, bram_msb/1, bram_lsb/1
